simulink model "Linear_2nd_order_model4Ident"  (R2024b)
settings: Solver=ode3  StartTime=0.0  StopTime=max(time)  FixedStep=T_sample  RelTol=1e-3  EnableMultiTasking=on
values from neighbouring files (symbols this model uses):
  a = -2*kesi* wn    (= -4.2)    [Linear_2nd_order_Sys_Model4Datacollection.m]    (also in Model_parameters_Ident.m = x_model(1))
  b = K*wn^2    (= 9)    [Linear_2nd_order_Sys_Model4Datacollection.m]    (also in Model_parameters_Ident.m = x_model(3))
  c = -wn^2    (= -9)    [Linear_2nd_order_Sys_Model4Datacollection.m]    (also in Model_parameters_Ident.m = x_model(2))
  f0 = 1    [Linear_2nd_order_Sys_Model4Datacollection.m]    (also in Model_parameters_Ident.m = x_model(4))
settings Model: Creator=shaocan  LastModifiedBy=sk3547969879
settings SolverCC: AlgebraicLoopSolver=TrustRegion
settings DataIOCC: LimitDataPoints=on  SaveFormat=Array  ReturnWorkspaceOutputs=off
settings OptimizationCC: LifeSpan=inf
settings DebuggingCC: UnconnectedInputMsg=warning  UnconnectedOutputMsg=warning  UnconnectedLineMsg=warning  SFUnexpectedBacktrackingDiag=warning  SFNoUnconditionalDefaultTransitionDiag=warning  SFExecutionAtInitializationDiag=none  ArithmeticOperatorsInVariantConditions=warning
settings HardwareCC: ProdBitPerPointer=32  ProdBitPerSizeT=32  ProdBitPerPtrDiffT=32  ProdLargestAtomicFloat=None  ProdIntDivRoundTo=Undefined  ProdEndianess=Unspecified  ProdWordSize=32  ProdHWDeviceType=32-bit Generic
settings ModelReferenceCC: EnableRefExpFcnMdlSchedulingChecks=on  PropagateSignalLabelsOutOfModel=off
settings SFSimCC: SimUseLocalCustomCode=off  CustomCodeUndefinedFunction=UseInterfaceOnly
settings RTWCC: RTWUseLocalCustomCode=off  GPUComputeCapability=3.5  DLArmComputeVersion=19.05
settings CodeAppCC: StateflowObjectComments=on
settings GRTTargetCC: TargetLangStandard=C89/C90 (ANSI)
settings ConfigComp: CovMetricSettings=dw  CovSaveCumulativeToWorkspaceVar=on  CovSaveSingleToWorkspaceVar=on  CovExternalEMLEnable=off  CovSFcnEnable=off

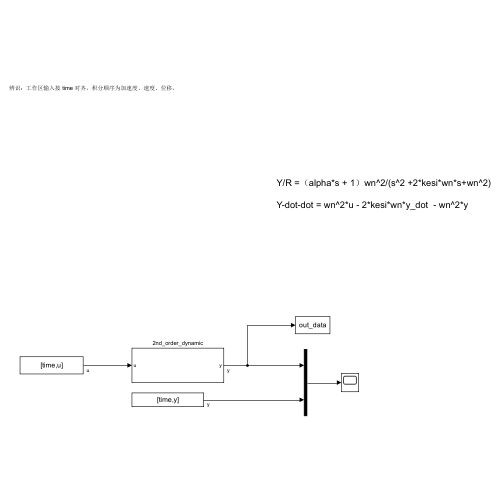
[thumbnail: Simulink's stored preview of the top-level diagram]
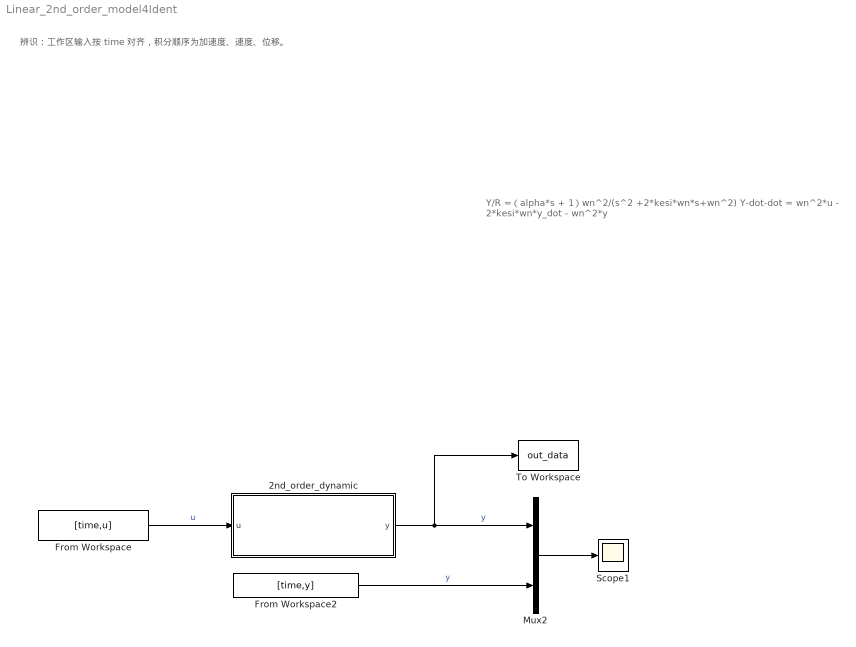
== system Linear_2nd_order_model4Ident ==
  note: Y/R =（alpha*s + 1）wn^2/(s^2 +2*kesi*wn*s+wn^2)
      |
      | Y-dot-dot = wn^2*u - 2*kesi*wn*y_dot - wn^2*y
  note: 辨识：工作区输入按 time 对齐，积分顺序为加速度、速度、位移。
  2nd_order_dynamic : Subsystem
  From Workspace : FromWorkspace  VariableName=[time,u]  Interpolate=off  OutputAfterFinalValue=Holding final value
  From Workspace2 : FromWorkspace  VariableName=[time,y]
  Mux2 : Mux  Inputs=2
  Scope1 : Scope
  To Workspace : ToWorkspace  VariableName=out_data  SaveFormat=Timeseries  SampleTime=-1
  wires:
  Mux2/1 -> Scope1/1
  From Workspace2/1 -> Mux2/2  "y"
  From Workspace/1 -> 2nd_order_dynamic/1(u)  "u"
  2nd_order_dynamic/1(y) -> To Workspace/1, Mux2/1  "y"

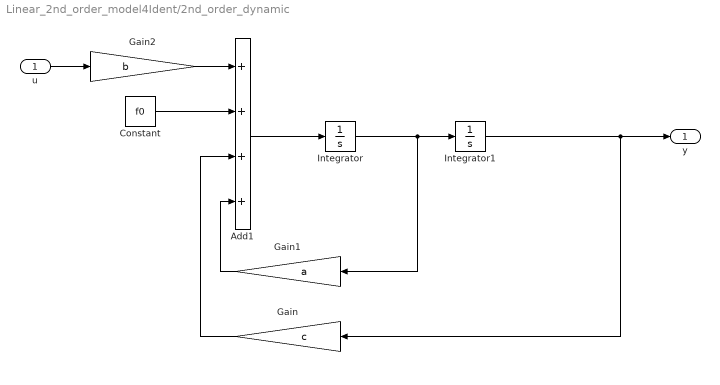
== system Linear_2nd_order_model4Ident/2nd_order_dynamic ==
  u : Inport
  Add1 : Sum  Inputs=++++
  Constant : Constant  Value=f0
  Gain : Gain  Gain=c
  Gain1 : Gain  Gain=a
  Gain2 : Gain  Gain=b
  Integrator : Integrator
  Integrator1 : Integrator
  y : Outport
  wires:
  Add1/1 -> Integrator/1
  Gain/1 -> Add1/3
  u/1 -> Gain2/1
  Integrator/1 -> Gain1/1, Integrator1/1
  Integrator1/1 -> Gain/1, y/1
  Gain2/1 -> Add1/1
  Gain1/1 -> Add1/4
  Constant/1 -> Add1/2
